simulink model "ah001_full_import"  (R2025b)
settings: Solver=VariableStepAuto  StartTime=0.0  StopTime=10.0  RelTol=1e-3
model workspace: external: MATLAB File C:\Users\Ben\Documents\GitHub\Bipedal_Robot\Neuromechanical_Models\AH001_Simscape_Repair\cad\export\ah001_full_DataFile.m (data not in the file)
undefined symbols (not defined in the file or in its folder): smiData, X, Y, Z
libraries: sm_lib x373, nesl_utility x1
(part 2 of 7)

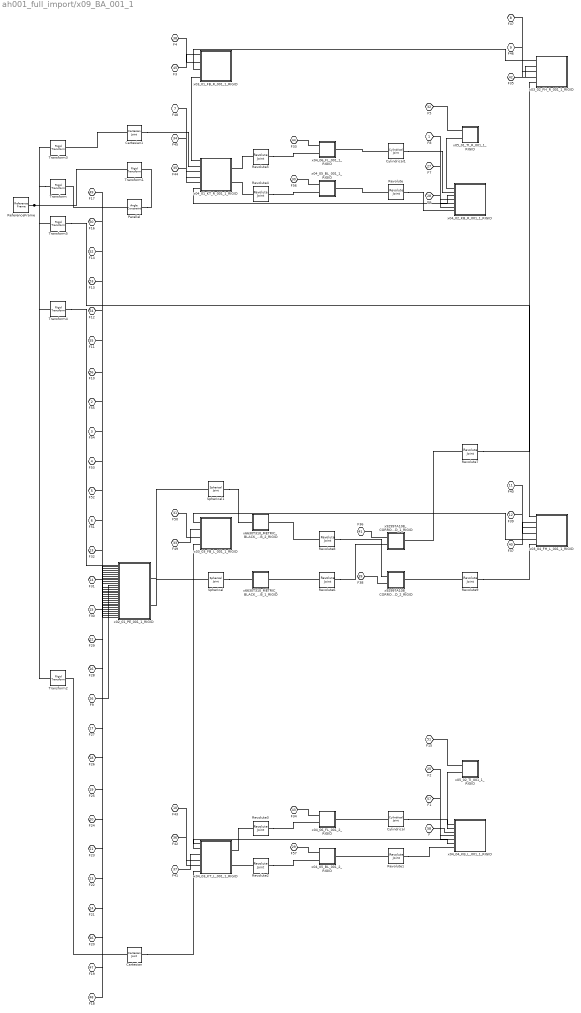
== system ah001_full_import/x09_BA_001_1 ==
  Cartesian : sm_lib/Joints/Cartesian Joint  JointMode=Normal  CompositeWrenchDir=FollowerOnBase  CompositeWrenchFrame=BaseFrame  SenseConstraintForce=off  SenseConstraintTorque=off  SenseTotalForce=off  SenseTotalTorque=off  PxPositionTargetSpecify=on  PxPositionTargetPriority=Low  PxPositionTargetValue=smiData.CartesianJoint(1).Px.Pos  PxPositionTargetValueUnits=m  PxVelocityTargetSpecify=off  PxVelocityTargetPriority=High  PxVelocityTargetValue=0  PxVelocityTargetValueUnits=m/s  PxEquilibriumPosition=0  PxEquilibriumPositionUnits=m  PxSpringStiffness=0  PxSpringStiffnessUnits=N/m  PxDampingCoefficient=0  PxDampingCoefficientUnits=N/(m/s)  PxLowerLimitSpecify=off  PxLowerLimitBound=-1  PxLowerLimitBoundUnits=m  PxLowerLimitStiffness=1e6  PxLowerLimitStiffnessUnits=N/m  PxLowerLimitDamping=1e3  PxLowerLimitDampingUnits=N/(m/s)  PxLowerLimitTransitionRegionWidth=1e-4  PxLowerLimitTransitionRegionWidthUnits=m  PxUpperLimitSpecify=off  PxUpperLimitBound=1  PxUpperLimitBoundUnits=m  PxUpperLimitStiffness=1e6  PxUpperLimitStiffnessUnits=N/m  PxUpperLimitDamping=1e3  PxUpperLimitDampingUnits=N/(m/s)  PxUpperLimitTransitionRegionWidth=1e-4  PxUpperLimitTransitionRegionWidthUnits=m  PxTorqueActuationMode=NoTorque  PxMotionActuationMode=ComputedMotion  PxSensePosition=off  PxSenseVelocity=off  PxSenseAcceleration=off  PxSenseTorqueForce=off  PxSenseLowerLimitTorqueForce=off  PxSenseUpperLimitTorqueForce=off  PyPositionTargetSpecify=on  PyPositionTargetPriority=Low  PyPositionTargetValue=smiData.CartesianJoint(1).Py.Pos  PyPositionTargetValueUnits=m  PyVelocityTargetSpecify=off  PyVelocityTargetPriority=High  PyVelocityTargetValue=0  PyVelocityTargetValueUnits=m/s  PyEquilibriumPosition=0  PyEquilibriumPositionUnits=m  PySpringStiffness=0  PySpringStiffnessUnits=N/m  PyDampingCoefficient=0  PyDampingCoefficientUnits=N/(m/s)  PyLowerLimitSpecify=off  PyLowerLimitBound=-1  PyLowerLimitBoundUnits=m  PyLowerLimitStiffness=1e6  PyLowerLimitStiffnessUnits=N/m  PyLowerLimitDamping=1e3  PyLowerLimitDampingUnits=N/(m/s)  PyLowerLimitTransitionRegionWidth=1e-4  PyLowerLimitTransitionRegionWidthUnits=m  PyUpperLimitSpecify=off  PyUpperLimitBound=1  PyUpperLimitBoundUnits=m  PyUpperLimitStiffness=1e6  PyUpperLimitStiffnessUnits=N/m  PyUpperLimitDamping=1e3  PyUpperLimitDampingUnits=N/(m/s)  PyUpperLimitTransitionRegionWidth=1e-4  PyUpperLimitTransitionRegionWidthUnits=m  PyTorqueActuationMode=NoTorque  PyMotionActuationMode=ComputedMotion  PySensePosition=off  PySenseVelocity=off  PySenseAcceleration=off  PySenseTorqueForce=off  PySenseLowerLimitTorqueForce=off  PySenseUpperLimitTorqueForce=off  PzPositionTargetSpecify=on  PzPositionTargetPriority=Low  PzPositionTargetValue=smiData.CartesianJoint(1).Pz.Pos  PzPositionTargetValueUnits=m  PzVelocityTargetSpecify=off  PzVelocityTargetPriority=High  PzVelocityTargetValue=0  PzVelocityTargetValueUnits=m/s  PzEquilibriumPosition=0  PzEquilibriumPositionUnits=m  PzSpringStiffness=0  PzSpringStiffnessUnits=N/m  PzDampingCoefficient=0  PzDampingCoefficientUnits=N/(m/s)  PzLowerLimitSpecify=off  PzLowerLimitBound=-1  PzLowerLimitBoundUnits=m  PzLowerLimitStiffness=1e6  PzLowerLimitStiffnessUnits=N/m  PzLowerLimitDamping=1e3  PzLowerLimitDampingUnits=N/(m/s)  PzLowerLimitTransitionRegionWidth=1e-4  PzLowerLimitTransitionRegionWidthUnits=m  PzUpperLimitSpecify=off  PzUpperLimitBound=1  PzUpperLimitBoundUnits=m  PzUpperLimitStiffness=1e6  PzUpperLimitStiffnessUnits=N/m  PzUpperLimitDamping=1e3  PzUpperLimitDampingUnits=N/(m/s)  PzUpperLimitTransitionRegionWidth=1e-4  PzUpperLimitTransitionRegionWidthUnits=m  PzTorqueActuationMode=NoTorque  PzMotionActuationMode=ComputedMotion  PzSensePosition=off  PzSenseVelocity=off  PzSenseAcceleration=off  PzSenseTorqueForce=off  PzSenseLowerLimitTorqueForce=off  PzSenseUpperLimitTorqueForce=off
  Cartesian1 : sm_lib/Joints/Cartesian Joint  JointMode=Normal  CompositeWrenchDir=FollowerOnBase  CompositeWrenchFrame=BaseFrame  SenseConstraintForce=off  SenseConstraintTorque=off  SenseTotalForce=off  SenseTotalTorque=off  PxPositionTargetSpecify=off  PxPositionTargetPriority=High  PxPositionTargetValue=0  PxPositionTargetValueUnits=m  PxVelocityTargetSpecify=off  PxVelocityTargetPriority=High  PxVelocityTargetValue=0  PxVelocityTargetValueUnits=m/s  PxEquilibriumPosition=0  PxEquilibriumPositionUnits=m  PxSpringStiffness=0  PxSpringStiffnessUnits=N/m  PxDampingCoefficient=0  PxDampingCoefficientUnits=N/(m/s)  PxLowerLimitSpecify=off  PxLowerLimitBound=-1  PxLowerLimitBoundUnits=m  PxLowerLimitStiffness=1e6  PxLowerLimitStiffnessUnits=N/m  PxLowerLimitDamping=1e3  PxLowerLimitDampingUnits=N/(m/s)  PxLowerLimitTransitionRegionWidth=1e-4  PxLowerLimitTransitionRegionWidthUnits=m  PxUpperLimitSpecify=off  PxUpperLimitBound=1  PxUpperLimitBoundUnits=m  PxUpperLimitStiffness=1e6  PxUpperLimitStiffnessUnits=N/m  PxUpperLimitDamping=1e3  PxUpperLimitDampingUnits=N/(m/s)  PxUpperLimitTransitionRegionWidth=1e-4  PxUpperLimitTransitionRegionWidthUnits=m  PxTorqueActuationMode=NoTorque  PxMotionActuationMode=ComputedMotion  PxSensePosition=off  PxSenseVelocity=off  PxSenseAcceleration=off  PxSenseTorqueForce=off  PxSenseLowerLimitTorqueForce=off  PxSenseUpperLimitTorqueForce=off  PyPositionTargetSpecify=off  PyPositionTargetPriority=High  PyPositionTargetValue=0  PyPositionTargetValueUnits=m  PyVelocityTargetSpecify=off  PyVelocityTargetPriority=High  PyVelocityTargetValue=0  PyVelocityTargetValueUnits=m/s  PyEquilibriumPosition=0  PyEquilibriumPositionUnits=m  PySpringStiffness=0  PySpringStiffnessUnits=N/m  PyDampingCoefficient=0  PyDampingCoefficientUnits=N/(m/s)  PyLowerLimitSpecify=off  PyLowerLimitBound=-1  PyLowerLimitBoundUnits=m  PyLowerLimitStiffness=1e6  PyLowerLimitStiffnessUnits=N/m  PyLowerLimitDamping=1e3  PyLowerLimitDampingUnits=N/(m/s)  PyLowerLimitTransitionRegionWidth=1e-4  PyLowerLimitTransitionRegionWidthUnits=m  PyUpperLimitSpecify=off  PyUpperLimitBound=1  PyUpperLimitBoundUnits=m  PyUpperLimitStiffness=1e6  PyUpperLimitStiffnessUnits=N/m  PyUpperLimitDamping=1e3  PyUpperLimitDampingUnits=N/(m/s)  PyUpperLimitTransitionRegionWidth=1e-4  PyUpperLimitTransitionRegionWidthUnits=m  PyTorqueActuationMode=NoTorque  PyMotionActuationMode=ComputedMotion  PySensePosition=off  PySenseVelocity=off  PySenseAcceleration=off  PySenseTorqueForce=off  PySenseLowerLimitTorqueForce=off  PySenseUpperLimitTorqueForce=off  PzPositionTargetSpecify=off  PzPositionTargetPriority=High  PzPositionTargetValue=0  PzPositionTargetValueUnits=m  PzVelocityTargetSpecify=off  PzVelocityTargetPriority=High  PzVelocityTargetValue=0  PzVelocityTargetValueUnits=m/s  PzEquilibriumPosition=0  PzEquilibriumPositionUnits=m  PzSpringStiffness=0  PzSpringStiffnessUnits=N/m  PzDampingCoefficient=0  PzDampingCoefficientUnits=N/(m/s)  PzLowerLimitSpecify=off  PzLowerLimitBound=-1  PzLowerLimitBoundUnits=m  PzLowerLimitStiffness=1e6  PzLowerLimitStiffnessUnits=N/m  PzLowerLimitDamping=1e3  PzLowerLimitDampingUnits=N/(m/s)  PzLowerLimitTransitionRegionWidth=1e-4  PzLowerLimitTransitionRegionWidthUnits=m  PzUpperLimitSpecify=off  PzUpperLimitBound=1  PzUpperLimitBoundUnits=m  PzUpperLimitStiffness=1e6  PzUpperLimitStiffnessUnits=N/m  PzUpperLimitDamping=1e3  PzUpperLimitDampingUnits=N/(m/s)  PzUpperLimitTransitionRegionWidth=1e-4  PzUpperLimitTransitionRegionWidthUnits=m  PzTorqueActuationMode=NoTorque  PzMotionActuationMode=ComputedMotion  PzSensePosition=off  PzSenseVelocity=off  PzSenseAcceleration=off  PzSenseTorqueForce=off  PzSenseLowerLimitTorqueForce=off  PzSenseUpperLimitTorqueForce=off
  Cylindrical : sm_lib/Joints/Cylindrical Joint  JointMode=Normal  CompositeWrenchDir=FollowerOnBase  CompositeWrenchFrame=BaseFrame  SenseConstraintForce=off  SenseConstraintTorque=off  SenseTotalForce=off  SenseTotalTorque=off  RzPositionTargetSpecify=off  RzPositionTargetPriority=High  RzPositionTargetValue=0  RzPositionTargetValueUnits=deg  RzVelocityTargetSpecify=off  RzVelocityTargetPriority=High  RzVelocityTargetValue=0  RzVelocityTargetValueUnits=deg/s  RzEquilibriumPosition=0  RzEquilibriumPositionUnits=deg  RzSpringStiffness=0  RzSpringStiffnessUnits=N*m/deg  RzDampingCoefficient=0  RzDampingCoefficientUnits=N*m/(deg/s)  RzLowerLimitSpecify=off  RzLowerLimitBound=-90  RzLowerLimitBoundUnits=deg  RzLowerLimitStiffness=1e4  RzLowerLimitStiffnessUnits=N*m/deg  RzLowerLimitDamping=10  RzLowerLimitDampingUnits=N*m/(deg/s)  RzLowerLimitTransitionRegionWidth=0.1  RzLowerLimitTransitionRegionWidthUnits=deg  RzUpperLimitSpecify=off  RzUpperLimitBound=90  RzUpperLimitBoundUnits=deg  RzUpperLimitStiffness=1e4  RzUpperLimitStiffnessUnits=N*m/deg  RzUpperLimitDamping=10  RzUpperLimitDampingUnits=N*m/(deg/s)  RzUpperLimitTransitionRegionWidth=0.1  RzUpperLimitTransitionRegionWidthUnits=deg  RzTorqueActuationMode=NoTorque  RzMotionActuationMode=ComputedMotion  RzSensePosition=off  RzSenseVelocity=off  RzSenseAcceleration=off  RzSenseTorqueForce=off  RzSenseLowerLimitTorqueForce=off  RzSenseUpperLimitTorqueForce=off  PzPositionTargetSpecify=off  PzPositionTargetPriority=High  PzPositionTargetValue=0  PzPositionTargetValueUnits=m  PzVelocityTargetSpecify=off  PzVelocityTargetPriority=High  PzVelocityTargetValue=0  PzVelocityTargetValueUnits=m/s  PzEquilibriumPosition=0  PzEquilibriumPositionUnits=m  PzSpringStiffness=0  PzSpringStiffnessUnits=N/m  PzDampingCoefficient=0  PzDampingCoefficientUnits=N/(m/s)  PzLowerLimitSpecify=off  PzLowerLimitBound=-1  PzLowerLimitBoundUnits=m  PzLowerLimitStiffness=1e6  PzLowerLimitStiffnessUnits=N/m  PzLowerLimitDamping=1e3  PzLowerLimitDampingUnits=N/(m/s)  PzLowerLimitTransitionRegionWidth=1e-4  PzLowerLimitTransitionRegionWidthUnits=m  PzUpperLimitSpecify=off  PzUpperLimitBound=1  PzUpperLimitBoundUnits=m  PzUpperLimitStiffness=1e6  PzUpperLimitStiffnessUnits=N/m  PzUpperLimitDamping=1e3  PzUpperLimitDampingUnits=N/(m/s)  PzUpperLimitTransitionRegionWidth=1e-4  PzUpperLimitTransitionRegionWidthUnits=m  PzTorqueActuationMode=NoTorque  PzMotionActuationMode=ComputedMotion  PzSensePosition=off  PzSenseVelocity=off  PzSenseAcceleration=off  PzSenseTorqueForce=off  PzSenseLowerLimitTorqueForce=off  PzSenseUpperLimitTorqueForce=off
  Cylindrical1 : sm_lib/Joints/Cylindrical Joint  JointMode=Normal  CompositeWrenchDir=FollowerOnBase  CompositeWrenchFrame=BaseFrame  SenseConstraintForce=off  SenseConstraintTorque=off  SenseTotalForce=off  SenseTotalTorque=off  RzPositionTargetSpecify=off  RzPositionTargetPriority=High  RzPositionTargetValue=0  RzPositionTargetValueUnits=deg  RzVelocityTargetSpecify=off  RzVelocityTargetPriority=High  RzVelocityTargetValue=0  RzVelocityTargetValueUnits=deg/s  RzEquilibriumPosition=0  RzEquilibriumPositionUnits=deg  RzSpringStiffness=0  RzSpringStiffnessUnits=N*m/deg  RzDampingCoefficient=0  RzDampingCoefficientUnits=N*m/(deg/s)  RzLowerLimitSpecify=off  RzLowerLimitBound=-90  RzLowerLimitBoundUnits=deg  RzLowerLimitStiffness=1e4  RzLowerLimitStiffnessUnits=N*m/deg  RzLowerLimitDamping=10  RzLowerLimitDampingUnits=N*m/(deg/s)  RzLowerLimitTransitionRegionWidth=0.1  RzLowerLimitTransitionRegionWidthUnits=deg  RzUpperLimitSpecify=off  RzUpperLimitBound=90  RzUpperLimitBoundUnits=deg  RzUpperLimitStiffness=1e4  RzUpperLimitStiffnessUnits=N*m/deg  RzUpperLimitDamping=10  RzUpperLimitDampingUnits=N*m/(deg/s)  RzUpperLimitTransitionRegionWidth=0.1  RzUpperLimitTransitionRegionWidthUnits=deg  RzTorqueActuationMode=NoTorque  RzMotionActuationMode=ComputedMotion  RzSensePosition=off  RzSenseVelocity=off  RzSenseAcceleration=off  RzSenseTorqueForce=off  RzSenseLowerLimitTorqueForce=off  RzSenseUpperLimitTorqueForce=off  PzPositionTargetSpecify=off  PzPositionTargetPriority=High  PzPositionTargetValue=0  PzPositionTargetValueUnits=m  PzVelocityTargetSpecify=off  PzVelocityTargetPriority=High  PzVelocityTargetValue=0  PzVelocityTargetValueUnits=m/s  PzEquilibriumPosition=0  PzEquilibriumPositionUnits=m  PzSpringStiffness=0  PzSpringStiffnessUnits=N/m  PzDampingCoefficient=0  PzDampingCoefficientUnits=N/(m/s)  PzLowerLimitSpecify=off  PzLowerLimitBound=-1  PzLowerLimitBoundUnits=m  PzLowerLimitStiffness=1e6  PzLowerLimitStiffnessUnits=N/m  PzLowerLimitDamping=1e3  PzLowerLimitDampingUnits=N/(m/s)  PzLowerLimitTransitionRegionWidth=1e-4  PzLowerLimitTransitionRegionWidthUnits=m  PzUpperLimitSpecify=off  PzUpperLimitBound=1  PzUpperLimitBoundUnits=m  PzUpperLimitStiffness=1e6  PzUpperLimitStiffnessUnits=N/m  PzUpperLimitDamping=1e3  PzUpperLimitDampingUnits=N/(m/s)  PzUpperLimitTransitionRegionWidth=1e-4  PzUpperLimitTransitionRegionWidthUnits=m  PzTorqueActuationMode=NoTorque  PzMotionActuationMode=ComputedMotion  PzSensePosition=off  PzSenseVelocity=off  PzSenseAcceleration=off  PzSenseTorqueForce=off  PzSenseLowerLimitTorqueForce=off  PzSenseUpperLimitTorqueForce=off
  Parallel : sm_lib/Constraints/Angle Constraint  ConstraintType=Parallel  Angle=45  AngleUnits=deg  WrenchDir=FollowerOnBase  WrenchFrame=BaseFrame  SenseTorque=off  SenseSignedTorqueMagnitude=off
  ReferenceFrame : sm_lib/Frames and Transforms/Reference Frame
  Revolute : sm_lib/Joints/Revolute Joint  JointMode=Normal  CompositeWrenchDir=FollowerOnBase  CompositeWrenchFrame=BaseFrame  SenseConstraintForce=off  SenseConstraintTorque=off  SenseTotalForce=off  SenseTotalTorque=off  PositionTargetSpecify=on  PositionTargetPriority=Low  PositionTargetValue=smiData.RevoluteJoint(1).Rz.Pos  PositionTargetValueUnits=deg  VelocityTargetSpecify=off  VelocityTargetPriority=High  VelocityTargetValue=0  VelocityTargetValueUnits=deg/s  EquilibriumPosition=0  EquilibriumPositionUnits=deg  SpringStiffness=0  SpringStiffnessUnits=N*m/deg  DampingCoefficient=0  DampingCoefficientUnits=N*m/(deg/s)  LowerLimitSpecify=off  LowerLimitBound=-90  LowerLimitBoundUnits=deg  LowerLimitStiffness=1e4  LowerLimitStiffnessUnits=N*m/deg  LowerLimitDamping=10  LowerLimitDampingUnits=N*m/(deg/s)  LowerLimitTransitionRegionWidth=0.1  LowerLimitTransitionRegionWidthUnits=deg  UpperLimitSpecify=off  UpperLimitBound=90  UpperLimitBoundUnits=deg  UpperLimitStiffness=1e4  UpperLimitStiffnessUnits=N*m/deg  UpperLimitDamping=10  UpperLimitDampingUnits=N*m/(deg/s)  UpperLimitTransitionRegionWidth=0.1  UpperLimitTransitionRegionWidthUnits=deg  TorqueActuationMode=NoTorque  MotionActuationMode=ComputedMotion  SensePosition=off  SenseVelocity=off  SenseAcceleration=off  SenseTorqueForce=off  SenseLowerLimitTorqueForce=off  SenseUpperLimitTorqueForce=off
  Revolute1 : sm_lib/Joints/Revolute Joint  JointMode=Normal  CompositeWrenchDir=FollowerOnBase  CompositeWrenchFrame=BaseFrame  SenseConstraintForce=off  SenseConstraintTorque=off  SenseTotalForce=off  SenseTotalTorque=off  PositionTargetSpecify=on  PositionTargetPriority=Low  PositionTargetValue=smiData.RevoluteJoint(2).Rz.Pos  PositionTargetValueUnits=deg  VelocityTargetSpecify=off  VelocityTargetPriority=High  VelocityTargetValue=0  VelocityTargetValueUnits=deg/s  EquilibriumPosition=0  EquilibriumPositionUnits=deg  SpringStiffness=0  SpringStiffnessUnits=N*m/deg  DampingCoefficient=0  DampingCoefficientUnits=N*m/(deg/s)  LowerLimitSpecify=off  LowerLimitBound=-90  LowerLimitBoundUnits=deg  LowerLimitStiffness=1e4  LowerLimitStiffnessUnits=N*m/deg  LowerLimitDamping=10  LowerLimitDampingUnits=N*m/(deg/s)  LowerLimitTransitionRegionWidth=0.1  LowerLimitTransitionRegionWidthUnits=deg  UpperLimitSpecify=off  UpperLimitBound=90  UpperLimitBoundUnits=deg  UpperLimitStiffness=1e4  UpperLimitStiffnessUnits=N*m/deg  UpperLimitDamping=10  UpperLimitDampingUnits=N*m/(deg/s)  UpperLimitTransitionRegionWidth=0.1  UpperLimitTransitionRegionWidthUnits=deg  TorqueActuationMode=NoTorque  MotionActuationMode=ComputedMotion  SensePosition=off  SenseVelocity=off  SenseAcceleration=off  SenseTorqueForce=off  SenseLowerLimitTorqueForce=off  SenseUpperLimitTorqueForce=off
  Revolute2 : sm_lib/Joints/Revolute Joint  JointMode=Normal  CompositeWrenchDir=FollowerOnBase  CompositeWrenchFrame=BaseFrame  SenseConstraintForce=off  SenseConstraintTorque=off  SenseTotalForce=off  SenseTotalTorque=off  PositionTargetSpecify=off  PositionTargetPriority=High  PositionTargetValue=0  PositionTargetValueUnits=deg  VelocityTargetSpecify=off  VelocityTargetPriority=High  VelocityTargetValue=0  VelocityTargetValueUnits=deg/s  EquilibriumPosition=0  EquilibriumPositionUnits=deg  SpringStiffness=0  SpringStiffnessUnits=N*m/deg  DampingCoefficient=0  DampingCoefficientUnits=N*m/(deg/s)  LowerLimitSpecify=off  LowerLimitBound=-90  LowerLimitBoundUnits=deg  LowerLimitStiffness=1e4  LowerLimitStiffnessUnits=N*m/deg  LowerLimitDamping=10  LowerLimitDampingUnits=N*m/(deg/s)  LowerLimitTransitionRegionWidth=0.1  LowerLimitTransitionRegionWidthUnits=deg  UpperLimitSpecify=off  UpperLimitBound=90  UpperLimitBoundUnits=deg  UpperLimitStiffness=1e4  UpperLimitStiffnessUnits=N*m/deg  UpperLimitDamping=10  UpperLimitDampingUnits=N*m/(deg/s)  UpperLimitTransitionRegionWidth=0.1  UpperLimitTransitionRegionWidthUnits=deg  TorqueActuationMode=NoTorque  MotionActuationMode=ComputedMotion  SensePosition=off  SenseVelocity=off  SenseAcceleration=off  SenseTorqueForce=off  SenseLowerLimitTorqueForce=off  SenseUpperLimitTorqueForce=off
  Revolute3 : sm_lib/Joints/Revolute Joint  JointMode=Normal  CompositeWrenchDir=FollowerOnBase  CompositeWrenchFrame=BaseFrame  SenseConstraintForce=off  SenseConstraintTorque=off  SenseTotalForce=off  SenseTotalTorque=off  PositionTargetSpecify=on  PositionTargetPriority=Low  PositionTargetValue=smiData.RevoluteJoint(4).Rz.Pos  PositionTargetValueUnits=deg  VelocityTargetSpecify=off  VelocityTargetPriority=High  VelocityTargetValue=0  VelocityTargetValueUnits=deg/s  EquilibriumPosition=0  EquilibriumPositionUnits=deg  SpringStiffness=0  SpringStiffnessUnits=N*m/deg  DampingCoefficient=0  DampingCoefficientUnits=N*m/(deg/s)  LowerLimitSpecify=off  LowerLimitBound=-90  LowerLimitBoundUnits=deg  LowerLimitStiffness=1e4  LowerLimitStiffnessUnits=N*m/deg  LowerLimitDamping=10  LowerLimitDampingUnits=N*m/(deg/s)  LowerLimitTransitionRegionWidth=0.1  LowerLimitTransitionRegionWidthUnits=deg  UpperLimitSpecify=off  UpperLimitBound=90  UpperLimitBoundUnits=deg  UpperLimitStiffness=1e4  UpperLimitStiffnessUnits=N*m/deg  UpperLimitDamping=10  UpperLimitDampingUnits=N*m/(deg/s)  UpperLimitTransitionRegionWidth=0.1  UpperLimitTransitionRegionWidthUnits=deg  TorqueActuationMode=NoTorque  MotionActuationMode=ComputedMotion  SensePosition=off  SenseVelocity=off  SenseAcceleration=off  SenseTorqueForce=off  SenseLowerLimitTorqueForce=off  SenseUpperLimitTorqueForce=off
  Revolute4 : sm_lib/Joints/Revolute Joint  JointMode=Normal  CompositeWrenchDir=FollowerOnBase  CompositeWrenchFrame=BaseFrame  SenseConstraintForce=off  SenseConstraintTorque=off  SenseTotalForce=off  SenseTotalTorque=off  PositionTargetSpecify=off  PositionTargetPriority=High  PositionTargetValue=0  PositionTargetValueUnits=deg  VelocityTargetSpecify=off  VelocityTargetPriority=High  VelocityTargetValue=0  VelocityTargetValueUnits=deg/s  EquilibriumPosition=0  EquilibriumPositionUnits=deg  SpringStiffness=0  SpringStiffnessUnits=N*m/deg  DampingCoefficient=0  DampingCoefficientUnits=N*m/(deg/s)  LowerLimitSpecify=off  LowerLimitBound=-90  LowerLimitBoundUnits=deg  LowerLimitStiffness=1e4  LowerLimitStiffnessUnits=N*m/deg  LowerLimitDamping=10  LowerLimitDampingUnits=N*m/(deg/s)  LowerLimitTransitionRegionWidth=0.1  LowerLimitTransitionRegionWidthUnits=deg  UpperLimitSpecify=off  UpperLimitBound=90  UpperLimitBoundUnits=deg  UpperLimitStiffness=1e4  UpperLimitStiffnessUnits=N*m/deg  UpperLimitDamping=10  UpperLimitDampingUnits=N*m/(deg/s)  UpperLimitTransitionRegionWidth=0.1  UpperLimitTransitionRegionWidthUnits=deg  TorqueActuationMode=NoTorque  MotionActuationMode=ComputedMotion  SensePosition=off  SenseVelocity=off  SenseAcceleration=off  SenseTorqueForce=off  SenseLowerLimitTorqueForce=off  SenseUpperLimitTorqueForce=off
  Revolute5 : sm_lib/Joints/Revolute Joint  JointMode=Normal  CompositeWrenchDir=FollowerOnBase  CompositeWrenchFrame=BaseFrame  SenseConstraintForce=off  SenseConstraintTorque=off  SenseTotalForce=off  SenseTotalTorque=off  PositionTargetSpecify=on  PositionTargetPriority=Low  PositionTargetValue=smiData.RevoluteJoint(6).Rz.Pos  PositionTargetValueUnits=deg  VelocityTargetSpecify=off  VelocityTargetPriority=High  VelocityTargetValue=0  VelocityTargetValueUnits=deg/s  EquilibriumPosition=0  EquilibriumPositionUnits=deg  SpringStiffness=0  SpringStiffnessUnits=N*m/deg  DampingCoefficient=0  DampingCoefficientUnits=N*m/(deg/s)  LowerLimitSpecify=off  LowerLimitBound=-90  LowerLimitBoundUnits=deg  LowerLimitStiffness=1e4  LowerLimitStiffnessUnits=N*m/deg  LowerLimitDamping=10  LowerLimitDampingUnits=N*m/(deg/s)  LowerLimitTransitionRegionWidth=0.1  LowerLimitTransitionRegionWidthUnits=deg  UpperLimitSpecify=off  UpperLimitBound=90  UpperLimitBoundUnits=deg  UpperLimitStiffness=1e4  UpperLimitStiffnessUnits=N*m/deg  UpperLimitDamping=10  UpperLimitDampingUnits=N*m/(deg/s)  UpperLimitTransitionRegionWidth=0.1  UpperLimitTransitionRegionWidthUnits=deg  TorqueActuationMode=NoTorque  MotionActuationMode=ComputedMotion  SensePosition=off  SenseVelocity=off  SenseAcceleration=off  SenseTorqueForce=off  SenseLowerLimitTorqueForce=off  SenseUpperLimitTorqueForce=off
  Revolute6 : sm_lib/Joints/Revolute Joint  JointMode=Normal  CompositeWrenchDir=FollowerOnBase  CompositeWrenchFrame=BaseFrame  SenseConstraintForce=off  SenseConstraintTorque=off  SenseTotalForce=off  SenseTotalTorque=off  PositionTargetSpecify=on  PositionTargetPriority=Low  PositionTargetValue=smiData.RevoluteJoint(7).Rz.Pos  PositionTargetValueUnits=deg  VelocityTargetSpecify=off  VelocityTargetPriority=High  VelocityTargetValue=0  VelocityTargetValueUnits=deg/s  EquilibriumPosition=0  EquilibriumPositionUnits=deg  SpringStiffness=0  SpringStiffnessUnits=N*m/deg  DampingCoefficient=0  DampingCoefficientUnits=N*m/(deg/s)  LowerLimitSpecify=off  LowerLimitBound=-90  LowerLimitBoundUnits=deg  LowerLimitStiffness=1e4  LowerLimitStiffnessUnits=N*m/deg  LowerLimitDamping=10  LowerLimitDampingUnits=N*m/(deg/s)  LowerLimitTransitionRegionWidth=0.1  LowerLimitTransitionRegionWidthUnits=deg  UpperLimitSpecify=off  UpperLimitBound=90  UpperLimitBoundUnits=deg  UpperLimitStiffness=1e4  UpperLimitStiffnessUnits=N*m/deg  UpperLimitDamping=10  UpperLimitDampingUnits=N*m/(deg/s)  UpperLimitTransitionRegionWidth=0.1  UpperLimitTransitionRegionWidthUnits=deg  TorqueActuationMode=NoTorque  MotionActuationMode=ComputedMotion  SensePosition=off  SenseVelocity=off  SenseAcceleration=off  SenseTorqueForce=off  SenseLowerLimitTorqueForce=off  SenseUpperLimitTorqueForce=off
  Revolute7 : sm_lib/Joints/Revolute Joint  JointMode=Normal  CompositeWrenchDir=FollowerOnBase  CompositeWrenchFrame=BaseFrame  SenseConstraintForce=off  SenseConstraintTorque=off  SenseTotalForce=off  SenseTotalTorque=off  PositionTargetSpecify=on  PositionTargetPriority=Low  PositionTargetValue=smiData.RevoluteJoint(8).Rz.Pos  PositionTargetValueUnits=deg  VelocityTargetSpecify=off  VelocityTargetPriority=High  VelocityTargetValue=0  VelocityTargetValueUnits=deg/s  EquilibriumPosition=0  EquilibriumPositionUnits=deg  SpringStiffness=0  SpringStiffnessUnits=N*m/deg  DampingCoefficient=0  DampingCoefficientUnits=N*m/(deg/s)  LowerLimitSpecify=off  LowerLimitBound=-90  LowerLimitBoundUnits=deg  LowerLimitStiffness=1e4  LowerLimitStiffnessUnits=N*m/deg  LowerLimitDamping=10  LowerLimitDampingUnits=N*m/(deg/s)  LowerLimitTransitionRegionWidth=0.1  LowerLimitTransitionRegionWidthUnits=deg  UpperLimitSpecify=off  UpperLimitBound=90  UpperLimitBoundUnits=deg  UpperLimitStiffness=1e4  UpperLimitStiffnessUnits=N*m/deg  UpperLimitDamping=10  UpperLimitDampingUnits=N*m/(deg/s)  UpperLimitTransitionRegionWidth=0.1  UpperLimitTransitionRegionWidthUnits=deg  TorqueActuationMode=NoTorque  MotionActuationMode=ComputedMotion  SensePosition=off  SenseVelocity=off  SenseAcceleration=off  SenseTorqueForce=off  SenseLowerLimitTorqueForce=off  SenseUpperLimitTorqueForce=off
  Revolute8 : sm_lib/Joints/Revolute Joint  JointMode=Normal  CompositeWrenchDir=FollowerOnBase  CompositeWrenchFrame=BaseFrame  SenseConstraintForce=off  SenseConstraintTorque=off  SenseTotalForce=off  SenseTotalTorque=off  PositionTargetSpecify=on  PositionTargetPriority=Low  PositionTargetValue=smiData.RevoluteJoint(9).Rz.Pos  PositionTargetValueUnits=deg  VelocityTargetSpecify=off  VelocityTargetPriority=High  VelocityTargetValue=0  VelocityTargetValueUnits=deg/s  EquilibriumPosition=0  EquilibriumPositionUnits=deg  SpringStiffness=0  SpringStiffnessUnits=N*m/deg  DampingCoefficient=0  DampingCoefficientUnits=N*m/(deg/s)  LowerLimitSpecify=off  LowerLimitBound=-90  LowerLimitBoundUnits=deg  LowerLimitStiffness=1e4  LowerLimitStiffnessUnits=N*m/deg  LowerLimitDamping=10  LowerLimitDampingUnits=N*m/(deg/s)  LowerLimitTransitionRegionWidth=0.1  LowerLimitTransitionRegionWidthUnits=deg  UpperLimitSpecify=off  UpperLimitBound=90  UpperLimitBoundUnits=deg  UpperLimitStiffness=1e4  UpperLimitStiffnessUnits=N*m/deg  UpperLimitDamping=10  UpperLimitDampingUnits=N*m/(deg/s)  UpperLimitTransitionRegionWidth=0.1  UpperLimitTransitionRegionWidthUnits=deg  TorqueActuationMode=NoTorque  MotionActuationMode=ComputedMotion  SensePosition=off  SenseVelocity=off  SenseAcceleration=off  SenseTorqueForce=off  SenseLowerLimitTorqueForce=off  SenseUpperLimitTorqueForce=off
  Revolute9 : sm_lib/Joints/Revolute Joint  JointMode=Normal  CompositeWrenchDir=FollowerOnBase  CompositeWrenchFrame=BaseFrame  SenseConstraintForce=off  SenseConstraintTorque=off  SenseTotalForce=off  SenseTotalTorque=off  PositionTargetSpecify=on  PositionTargetPriority=Low  PositionTargetValue=smiData.RevoluteJoint(10).Rz.Pos  PositionTargetValueUnits=deg  VelocityTargetSpecify=off  VelocityTargetPriority=High  VelocityTargetValue=0  VelocityTargetValueUnits=deg/s  EquilibriumPosition=0  EquilibriumPositionUnits=deg  SpringStiffness=0  SpringStiffnessUnits=N*m/deg  DampingCoefficient=0  DampingCoefficientUnits=N*m/(deg/s)  LowerLimitSpecify=off  LowerLimitBound=-90  LowerLimitBoundUnits=deg  LowerLimitStiffness=1e4  LowerLimitStiffnessUnits=N*m/deg  LowerLimitDamping=10  LowerLimitDampingUnits=N*m/(deg/s)  LowerLimitTransitionRegionWidth=0.1  LowerLimitTransitionRegionWidthUnits=deg  UpperLimitSpecify=off  UpperLimitBound=90  UpperLimitBoundUnits=deg  UpperLimitStiffness=1e4  UpperLimitStiffnessUnits=N*m/deg  UpperLimitDamping=10  UpperLimitDampingUnits=N*m/(deg/s)  UpperLimitTransitionRegionWidth=0.1  UpperLimitTransitionRegionWidthUnits=deg  TorqueActuationMode=NoTorque  MotionActuationMode=ComputedMotion  SensePosition=off  SenseVelocity=off  SenseAcceleration=off  SenseTorqueForce=off  SenseLowerLimitTorqueForce=off  SenseUpperLimitTorqueForce=off
  Spherical : sm_lib/Joints/Spherical Joint  JointMode=Normal  CompositeWrenchDir=FollowerOnBase  CompositeWrenchFrame=BaseFrame  SenseConstraintForce=off  SenseConstraintTorque=off  SenseTotalForce=off  SenseTotalTorque=off  PositionTargetSpecify=on  PositionTargetPriority=Low  PositionTargetRotationMethod=ArbitraryAxis  PositionTargetFollAlignAxisA=+X  PositionTargetBaseAlignAxisA=+Y  PositionTargetFollAlignAxisB=+Y  PositionTargetBaseAlignAxisB=+Z  PositionTargetRotationStandardAxis=+Z  PositionTargetRotationAngle=smiData.SphericalJoint(1).S.Pos.Angle  PositionTargetRotationAngleUnits=deg  PositionTargetRotationArbitraryAxis=smiData.SphericalJoint(1).S.Pos.Axis  PositionTargetRotationSequenceAxes=FollowerAxes  PositionTargetRotationSequence=XYX  PositionTargetRotationSequenceAngles=[0 0 0]  PositionTargetRotationSequenceAnglesUnits=deg  PositionTargetRotationMatrix=[1 0 0;0 1 0;0 0 1]  PositionTargetQuaternion=[1 0 0 0]  VelocityTargetSpecify=off  VelocityTargetPriority=High  VelocityTargetValue=[0 0 0]  VelocityTargetValueUnits=deg/s  VelocityTargetInFollowerFrame=on  EqPosRotationMethod=None  EqPosFollAlignAxisA=+X  EqPosBaseAlignAxisA=+Y  EqPosFollAlignAxisB=+Y  EqPosBaseAlignAxisB=+Z  EqPosRotationStandardAxis=+Z  EqPosRotationAngle=0  EqPosRotationAngleUnits=deg  EqPosRotationArbitraryAxis=[0 0 1]  EqPosRotationSequenceAxes=FollowerAxes  EqPosRotationSequence=XYX  EqPosRotationSequenceAngles=[0 0 0]  EqPosRotationSequenceAnglesUnits=deg  EqPosRotationMatrix=[1 0 0;0 1 0;0 0 1]  EqPosQuaternion=[1 0 0 0]  SpringStiffness=0  SpringStiffnessUnits=N*m/deg  DampingCoefficient=0  DampingCoefficientUnits=N*m/(deg/s)  LowerLimitSpecify=off  LowerLimitBound=15  LowerLimitBoundUnits=deg  LowerLimitStiffness=1e4  LowerLimitStiffnessUnits=N*m/deg  LowerLimitDamping=10  LowerLimitDampingUnits=N*m/(deg/s)  LowerLimitTransitionRegionWidth=0.1  LowerLimitTransitionRegionWidthUnits=deg  UpperLimitSpecify=off  UpperLimitBound=45  UpperLimitBoundUnits=deg  UpperLimitStiffness=1e4  UpperLimitStiffnessUnits=N*m/deg  UpperLimitDamping=10  UpperLimitDampingUnits=N*m/(deg/s)  UpperLimitTransitionRegionWidth=0.1  UpperLimitTransitionRegionWidthUnits=deg  TorqueActuationMode=NoTorque  ActuateTorqueX=off  ActuateTorqueY=off  ActuateTorqueZ=off  ActuateTorque=off  ActuationFrame=BaseFrame  SensePosition=off  SenseVelocityX=off  SenseVelocityY=off  SenseVelocityZ=off  SenseVelocity=off  SenseAccelerationX=off  SenseAccelerationY=off  SenseAccelerationZ=off  SenseAcceleration=off  SenseLowerLimitTorqueMag=off  SenseUpperLimitTorqueMag=off  SensingFrame=FollowerFrame
  Spherical1 : sm_lib/Joints/Spherical Joint  JointMode=Normal  CompositeWrenchDir=FollowerOnBase  CompositeWrenchFrame=BaseFrame  SenseConstraintForce=off  SenseConstraintTorque=off  SenseTotalForce=off  SenseTotalTorque=off  PositionTargetSpecify=off  PositionTargetPriority=High  PositionTargetRotationMethod=None  PositionTargetFollAlignAxisA=+X  PositionTargetBaseAlignAxisA=+Y  PositionTargetFollAlignAxisB=+Y  PositionTargetBaseAlignAxisB=+Z  PositionTargetRotationStandardAxis=+Z  PositionTargetRotationAngle=0  PositionTargetRotationAngleUnits=deg  PositionTargetRotationArbitraryAxis=[0 0 1]  PositionTargetRotationSequenceAxes=FollowerAxes  PositionTargetRotationSequence=XYX  PositionTargetRotationSequenceAngles=[0 0 0]  PositionTargetRotationSequenceAnglesUnits=deg  PositionTargetRotationMatrix=[1 0 0;0 1 0;0 0 1]  PositionTargetQuaternion=[1 0 0 0]  VelocityTargetSpecify=off  VelocityTargetPriority=High  VelocityTargetValue=[0 0 0]  VelocityTargetValueUnits=deg/s  VelocityTargetInFollowerFrame=on  EqPosRotationMethod=None  EqPosFollAlignAxisA=+X  EqPosBaseAlignAxisA=+Y  EqPosFollAlignAxisB=+Y  EqPosBaseAlignAxisB=+Z  EqPosRotationStandardAxis=+Z  EqPosRotationAngle=0  EqPosRotationAngleUnits=deg  EqPosRotationArbitraryAxis=[0 0 1]  EqPosRotationSequenceAxes=FollowerAxes  EqPosRotationSequence=XYX  EqPosRotationSequenceAngles=[0 0 0]  EqPosRotationSequenceAnglesUnits=deg  EqPosRotationMatrix=[1 0 0;0 1 0;0 0 1]  EqPosQuaternion=[1 0 0 0]  SpringStiffness=0  SpringStiffnessUnits=N*m/deg  DampingCoefficient=0  DampingCoefficientUnits=N*m/(deg/s)  LowerLimitSpecify=off  LowerLimitBound=15  LowerLimitBoundUnits=deg  LowerLimitStiffness=1e4  LowerLimitStiffnessUnits=N*m/deg  LowerLimitDamping=10  LowerLimitDampingUnits=N*m/(deg/s)  LowerLimitTransitionRegionWidth=0.1  LowerLimitTransitionRegionWidthUnits=deg  UpperLimitSpecify=off  UpperLimitBound=45  UpperLimitBoundUnits=deg  UpperLimitStiffness=1e4  UpperLimitStiffnessUnits=N*m/deg  UpperLimitDamping=10  UpperLimitDampingUnits=N*m/(deg/s)  UpperLimitTransitionRegionWidth=0.1  UpperLimitTransitionRegionWidthUnits=deg  TorqueActuationMode=NoTorque  ActuateTorqueX=off  ActuateTorqueY=off  ActuateTorqueZ=off  ActuateTorque=off  ActuationFrame=BaseFrame  SensePosition=off  SenseVelocityX=off  SenseVelocityY=off  SenseVelocityZ=off  SenseVelocity=off  SenseAccelerationX=off  SenseAccelerationY=off  SenseAccelerationZ=off  SenseAcceleration=off  SenseLowerLimitTorqueMag=off  SenseUpperLimitTorqueMag=off  SensingFrame=FollowerFrame
  Transform : sm_lib/Frames and Transforms/Rigid Transform  RotationMethod=ArbitraryAxis  FollAlignAxisA=+X  BaseAlignAxisA=+Y  FollAlignAxisB=+Y  BaseAlignAxisB=+Z  RotationStandardAxis=+Z  RotationAngle=smiData.RigidTransform(21).angle  RotationAngleUnits=rad  RotationArbitraryAxis=smiData.RigidTransform(21).axis  RotationSequenceAxes=FollowerAxes  RotationSequence=XYX  RotationSequenceAngles=[0 0 0]  RotationSequenceAnglesUnits=deg  RotationMatrix=[1 0 0;0 1 0;0 0 1]  Quaternion=[1 0 0 0]  TranslationMethod=Cartesian  TranslationCartesianOffset=smiData.RigidTransform(21).translation  TranslationCartesianOffsetUnits=mm  TranslationStandardAxis=+Z  TranslationStandardOffset=0  TranslationStandardOffsetUnits=m  TranslationROffset=0  TranslationROffsetUnits=m  TranslationThetaOffset=0  TranslationThetaOffsetUnits=deg  TranslationZOffset=0  TranslationZOffsetUnits=m
  Transform1 : sm_lib/Frames and Transforms/Rigid Transform  RotationMethod=ArbitraryAxis  FollAlignAxisA=+X  BaseAlignAxisA=+Y  FollAlignAxisB=+Y  BaseAlignAxisB=+Z  RotationStandardAxis=+Z  RotationAngle=smiData.RigidTransform(22).angle  RotationAngleUnits=rad  RotationArbitraryAxis=smiData.RigidTransform(22).axis  RotationSequenceAxes=FollowerAxes  RotationSequence=XYX  RotationSequenceAngles=[0 0 0]  RotationSequenceAnglesUnits=deg  RotationMatrix=[1 0 0;0 1 0;0 0 1]  Quaternion=[1 0 0 0]  TranslationMethod=Cartesian  TranslationCartesianOffset=smiData.RigidTransform(22).translation  TranslationCartesianOffsetUnits=mm  TranslationStandardAxis=+Z  TranslationStandardOffset=0  TranslationStandardOffsetUnits=m  TranslationROffset=0  TranslationROffsetUnits=m  TranslationThetaOffset=0  TranslationThetaOffsetUnits=deg  TranslationZOffset=0  TranslationZOffsetUnits=m
  Transform2 : sm_lib/Frames and Transforms/Rigid Transform  RotationMethod=ArbitraryAxis  FollAlignAxisA=+X  BaseAlignAxisA=+Y  FollAlignAxisB=+Y  BaseAlignAxisB=+Z  RotationStandardAxis=+Z  RotationAngle=smiData.RigidTransform(23).angle  RotationAngleUnits=rad  RotationArbitraryAxis=smiData.RigidTransform(23).axis  RotationSequenceAxes=FollowerAxes  RotationSequence=XYX  RotationSequenceAngles=[0 0 0]  RotationSequenceAnglesUnits=deg  RotationMatrix=[1 0 0;0 1 0;0 0 1]  Quaternion=[1 0 0 0]  TranslationMethod=Cartesian  TranslationCartesianOffset=smiData.RigidTransform(23).translation  TranslationCartesianOffsetUnits=mm  TranslationStandardAxis=+Z  TranslationStandardOffset=0  TranslationStandardOffsetUnits=m  TranslationROffset=0  TranslationROffsetUnits=m  TranslationThetaOffset=0  TranslationThetaOffsetUnits=deg  TranslationZOffset=0  TranslationZOffsetUnits=m
  Transform3 : sm_lib/Frames and Transforms/Rigid Transform  RotationMethod=ArbitraryAxis  FollAlignAxisA=+X  BaseAlignAxisA=+Y  FollAlignAxisB=+Y  BaseAlignAxisB=+Z  RotationStandardAxis=+Z  RotationAngle=smiData.RigidTransform(37).angle  RotationAngleUnits=rad  RotationArbitraryAxis=smiData.RigidTransform(37).axis  RotationSequenceAxes=FollowerAxes  RotationSequence=XYX  RotationSequenceAngles=[0 0 0]  RotationSequenceAnglesUnits=deg  RotationMatrix=[1 0 0;0 1 0;0 0 1]  Quaternion=[1 0 0 0]  TranslationMethod=Cartesian  TranslationCartesianOffset=smiData.RigidTransform(37).translation  TranslationCartesianOffsetUnits=mm  TranslationStandardAxis=+Z  TranslationStandardOffset=0  TranslationStandardOffsetUnits=m  TranslationROffset=0  TranslationROffsetUnits=m  TranslationThetaOffset=0  TranslationThetaOffsetUnits=deg  TranslationZOffset=0  TranslationZOffsetUnits=m
  Transform4 : sm_lib/Frames and Transforms/Rigid Transform  RotationMethod=ArbitraryAxis  FollAlignAxisA=+X  BaseAlignAxisA=+Y  FollAlignAxisB=+Y  BaseAlignAxisB=+Z  RotationStandardAxis=+Z  RotationAngle=smiData.RigidTransform(167).angle  RotationAngleUnits=rad  RotationArbitraryAxis=smiData.RigidTransform(167).axis  RotationSequenceAxes=FollowerAxes  RotationSequence=XYX  RotationSequenceAngles=[0 0 0]  RotationSequenceAnglesUnits=deg  RotationMatrix=[1 0 0;0 1 0;0 0 1]  Quaternion=[1 0 0 0]  TranslationMethod=Cartesian  TranslationCartesianOffset=smiData.RigidTransform(167).translation  TranslationCartesianOffsetUnits=mm  TranslationStandardAxis=+Z  TranslationStandardOffset=0  TranslationStandardOffsetUnits=m  TranslationROffset=0  TranslationROffsetUnits=m  TranslationThetaOffset=0  TranslationThetaOffsetUnits=deg  TranslationZOffset=0  TranslationZOffsetUnits=m
  Transform5 : sm_lib/Frames and Transforms/Rigid Transform  RotationMethod=ArbitraryAxis  FollAlignAxisA=+X  BaseAlignAxisA=+Y  FollAlignAxisB=+Y  BaseAlignAxisB=+Z  RotationStandardAxis=+Z  RotationAngle=smiData.RigidTransform(168).angle  RotationAngleUnits=rad  RotationArbitraryAxis=smiData.RigidTransform(168).axis  RotationSequenceAxes=FollowerAxes  RotationSequence=XYX  RotationSequenceAngles=[0 0 0]  RotationSequenceAnglesUnits=deg  RotationMatrix=[1 0 0;0 1 0;0 0 1]  Quaternion=[1 0 0 0]  TranslationMethod=Cartesian  TranslationCartesianOffset=smiData.RigidTransform(168).translation  TranslationCartesianOffsetUnits=mm  TranslationStandardAxis=+Z  TranslationStandardOffset=0  TranslationStandardOffsetUnits=m  TranslationROffset=0  TranslationROffsetUnits=m  TranslationThetaOffset=0  TranslationThetaOffsetUnits=deg  TranslationZOffset=0  TranslationZOffsetUnits=m
  x02_01_PE_001_1_RIGID : Subsystem
  x03_01_FB_R_001_1_RIGID : Subsystem
  x03_02_FH_R_001_1_RIGID : Subsystem
  x03_03_FB_L_001_1_RIGID : Subsystem
  x03_04_FH_L_001_1_RIGID : Subsystem
  x04_01_KT_R_001_1_RIGID : Subsystem
  x04_02_KB_R_001_1_RIGID : Subsystem
  x04_03_KT_L_001_1_RIGID : Subsystem
  x04_04_KB_L_001_1_RIGID : Subsystem
  x04_05_BL_001_1_RIGID : Subsystem
  x04_05_BL_001_2_RIGID : Subsystem
  x04_06_FL_001_1_RIGID : Subsystem
  x04_06_FL_001_2_RIGID : Subsystem
  x05_01_TI_R_001_1_RIGID : Subsystem
  x05_02_TI_001_1_RIGID : Subsystem
  x6630T310_METRIC_BLACK_POLYPROPYLENE_BALL_KNOB_1_RIGID : Subsystem
  x6630T310_METRIC_BLACK_POLYPROPYLENE_BALL_KNOB_2_RIGID : Subsystem
  x92997A108_CORROSION_RESISTANT_SETUP_STUD_1_RIGID : Subsystem
  x92997A108_CORROSION_RESISTANT_SETUP_STUD_2_RIGID : Subsystem
  F8 : PMIOPort  Side=Left
  F55 : PMIOPort  Port=2  Side=Left
  F54 : PMIOPort  Port=3  Side=Left
  F53 : PMIOPort  Port=4  Side=Left
  F52 : PMIOPort  Port=5  Side=Left
  F51 : PMIOPort  Port=6  Side=Left
  F48 : PMIOPort  Port=7  Side=Left
  F47 : PMIOPort  Port=8  Side=Left
  F46 : PMIOPort  Port=9  Side=Left
  F43 : PMIOPort  Port=10  Side=Left
  F40 : PMIOPort  Port=11  Side=Left
  F39 : PMIOPort  Port=12  Side=Left
  F32 : PMIOPort  Port=13  Side=Left
  F31 : PMIOPort  Port=14  Side=Left
  F30 : PMIOPort  Port=15  Side=Left
  F28 : PMIOPort  Port=16  Side=Left
  F27 : PMIOPort  Port=17  Side=Left
  F26 : PMIOPort  Port=18  Side=Left
  F25 : PMIOPort  Port=19  Side=Left
  F24 : PMIOPort  Port=20  Side=Left
  F23 : PMIOPort  Port=21  Side=Left
  F29 : PMIOPort  Port=22  Side=Left
  F22 : PMIOPort  Port=23  Side=Left
  F21 : PMIOPort  Port=24  Side=Left
  F2 : PMIOPort  Port=25  Side=Left
  F9 : PMIOPort  Port=26  Side=Right
  F7 : PMIOPort  Port=27  Side=Right
  F6 : PMIOPort  Port=28  Side=Right
  F57 : PMIOPort  Port=29  Side=Right
  F56 : PMIOPort  Port=30  Side=Right
  F50 : PMIOPort  Port=31  Side=Right
  F5 : PMIOPort  Port=32  Side=Right
  F49 : PMIOPort  Port=33  Side=Right
  F45 : PMIOPort  Port=34  Side=Right
  F44 : PMIOPort  Port=35  Side=Right
  F42 : PMIOPort  Port=36  Side=Right
  F41 : PMIOPort  Port=37  Side=Right
  F4 : PMIOPort  Port=38  Side=Right
  F38 : PMIOPort  Port=39  Side=Right
  F37 : PMIOPort  Port=40  Side=Right
  F36 : PMIOPort  Port=41  Side=Right
  F35 : PMIOPort  Port=42  Side=Right
  F34 : PMIOPort  Port=43  Side=Right
  F33 : PMIOPort  Port=44  Side=Right
  F3 : PMIOPort  Port=45  Side=Right
  F20 : PMIOPort  Port=46  Side=Right
  F19 : PMIOPort  Port=47  Side=Right
  F18 : PMIOPort  Port=48  Side=Right
  F17 : PMIOPort  Port=49  Side=Right
  F16 : PMIOPort  Port=50  Side=Right
  F15 : PMIOPort  Port=51  Side=Right
  F14 : PMIOPort  Port=52  Side=Right
  F13 : PMIOPort  Port=53  Side=Right
  F12 : PMIOPort  Port=54  Side=Right
  F11 : PMIOPort  Port=55  Side=Right
  F10 : PMIOPort  Port=56  Side=Right
  F1 : PMIOPort  Port=57  Side=Right
  F : PMIOPort  Port=58  Side=Right
  connections:
  Revolute/LConn1 -- x04_05_BL_001_1_RIGID/RConn1
  Revolute/RConn1 -- x04_02_KB_R_001_1_RIGID/LConn7
  Spherical/RConn1 -- x6630T310_METRIC_BLACK_POLYPROPYLENE_BALL_KNOB_1_RIGID/LConn1
  x04_05_BL_001_2_RIGID/LConn1 -- F57/RConn1
  Transform4/RConn1 -- x02_01_PE_001_1_RIGID/LConn1
  Transform5/RConn1 -- x03_04_FH_L_001_1_RIGID/LConn1
  Spherical1/LConn1 -- x02_01_PE_001_1_RIGID/RConn1
  Spherical1/RConn1 -- x6630T310_METRIC_BLACK_POLYPROPYLENE_BALL_KNOB_2_RIGID/LConn1
  Cylindrical/LConn1 -- x04_06_FL_001_2_RIGID/RConn1
  Cylindrical/RConn1 -- x04_04_KB_L_001_1_RIGID/LConn2
  x04_03_KT_L_001_1_RIGID/LConn2 -- x04_04_KB_L_001_1_RIGID/LConn6
  Transform/LConn1 -- ReferenceFrame/RConn1 -- Transform1/LConn1 -- Transform2/LConn1 -- Transform3/LConn1 -- Transform4/LConn1 -- Transform5/LConn1
  Parallel/LConn1 -- Transform/RConn1
  Parallel/RConn1 -- Transform1/RConn1
  Cartesian/LConn1 -- Transform2/RConn1
  Revolute1/LConn1 -- x04_05_BL_001_2_RIGID/RConn1
  Cartesian/RConn1 -- x04_03_KT_L_001_1_RIGID/LConn6
  x04_02_KB_R_001_1_RIGID/LConn1 -- x05_01_TI_R_001_1_RIGID/LConn2
  Cylindrical1/LConn1 -- x04_06_FL_001_1_RIGID/RConn1
  Cylindrical1/RConn1 -- x04_02_KB_R_001_1_RIGID/LConn2
  Revolute3/LConn1 -- x04_03_KT_L_001_1_RIGID/RConn1
  Revolute3/RConn1 -- x04_06_FL_001_2_RIGID/LConn2
  x03_01_FB_R_001_1_RIGID/LConn3 -- x03_02_FH_R_001_1_RIGID/LConn1
  Revolute4/LConn1 -- x04_01_KT_R_001_1_RIGID/RConn2
  Revolute4/RConn1 -- x04_05_BL_001_1_RIGID/LConn2
  x03_01_FB_R_001_1_RIGID/LConn4 -- x04_01_KT_R_001_1_RIGID/LConn1
  Revolute1/RConn1 -- x04_04_KB_L_001_1_RIGID/LConn7
  Cartesian1/LConn1 -- Transform3/RConn1
  Cartesian1/RConn1 -- x04_01_KT_R_001_1_RIGID/LConn2
  x04_01_KT_R_001_1_RIGID/LConn6 -- x04_02_KB_R_001_1_RIGID/LConn3
  Revolute5/LConn1 -- x04_01_KT_R_001_1_RIGID/RConn1
  Revolute5/RConn1 -- x04_06_FL_001_1_RIGID/LConn2
  Revolute6/LConn1 -- x6630T310_METRIC_BLACK_POLYPROPYLENE_BALL_KNOB_1_RIGID/RConn1
  Revolute6/RConn1 -- x92997A108_CORROSION_RESISTANT_SETUP_STUD_1_RIGID/LConn2
  Revolute7/LConn1 -- x92997A108_CORROSION_RESISTANT_SETUP_STUD_1_RIGID/RConn1
  Revolute7/RConn1 -- x03_02_FH_R_001_1_RIGID/LConn5
  Revolute8/LConn1 -- x6630T310_METRIC_BLACK_POLYPROPYLENE_BALL_KNOB_2_RIGID/RConn1
  Revolute2/LConn1 -- x04_03_KT_L_001_1_RIGID/RConn2
  Revolute8/RConn1 -- x92997A108_CORROSION_RESISTANT_SETUP_STUD_2_RIGID/LConn1
  Revolute9/LConn1 -- x92997A108_CORROSION_RESISTANT_SETUP_STUD_2_RIGID/RConn1
  Revolute9/RConn1 -- x03_04_FH_L_001_1_RIGID/LConn6
  x04_04_KB_L_001_1_RIGID/LConn3 -- F/RConn1
  x04_04_KB_L_001_1_RIGID/LConn4 -- F1/RConn1
  x04_04_KB_L_001_1_RIGID/LConn5 -- F2/RConn1
  x03_01_FB_R_001_1_RIGID/LConn1 -- F3/RConn1
  x03_01_FB_R_001_1_RIGID/LConn2 -- F4/RConn1
  x05_01_TI_R_001_1_RIGID/LConn1 -- F5/RConn1
  x04_02_KB_R_001_1_RIGID/LConn4 -- F6/RConn1
  Revolute2/RConn1 -- x04_05_BL_001_2_RIGID/LConn2
  x04_02_KB_R_001_1_RIGID/LConn5 -- F7/RConn1
  x04_02_KB_R_001_1_RIGID/LConn6 -- F8/RConn1
  x02_01_PE_001_1_RIGID/LConn12 -- F9/RConn1
  x02_01_PE_001_1_RIGID/LConn23 -- F10/RConn1
  x02_01_PE_001_1_RIGID/LConn24 -- F11/RConn1
  x02_01_PE_001_1_RIGID/LConn25 -- F12/RConn1
  x02_01_PE_001_1_RIGID/LConn26 -- F13/RConn1
  x02_01_PE_001_1_RIGID/LConn27 -- F14/RConn1
  x05_02_TI_001_1_RIGID/LConn1 -- F15/RConn1
  x02_01_PE_001_1_RIGID/LConn28 -- F16/RConn1
  x03_03_FB_L_001_1_RIGID/LConn1 -- x03_04_FH_L_001_1_RIGID/LConn5
  x02_01_PE_001_1_RIGID/LConn29 -- F17/RConn1
  x02_01_PE_001_1_RIGID/LConn2 -- F18/RConn1
  x02_01_PE_001_1_RIGID/LConn3 -- F19/RConn1
  x02_01_PE_001_1_RIGID/LConn4 -- F20/RConn1
  x02_01_PE_001_1_RIGID/LConn5 -- F21/RConn1
  x02_01_PE_001_1_RIGID/LConn6 -- F22/RConn1
  x02_01_PE_001_1_RIGID/LConn7 -- F23/RConn1
  x02_01_PE_001_1_RIGID/LConn8 -- F24/RConn1
  x02_01_PE_001_1_RIGID/LConn9 -- F25/RConn1
  x02_01_PE_001_1_RIGID/LConn10 -- F26/RConn1
  x03_03_FB_L_001_1_RIGID/LConn4 -- x04_03_KT_L_001_1_RIGID/LConn1
  x02_01_PE_001_1_RIGID/LConn11 -- F27/RConn1
  x02_01_PE_001_1_RIGID/LConn13 -- F28/RConn1
  x02_01_PE_001_1_RIGID/LConn14 -- F29/RConn1
  x02_01_PE_001_1_RIGID/LConn15 -- F30/RConn1
  x02_01_PE_001_1_RIGID/LConn16 -- F31/RConn1
  x02_01_PE_001_1_RIGID/LConn17 -- F32/RConn1
  x04_06_FL_001_1_RIGID/LConn1 -- F33/RConn1
  x04_06_FL_001_2_RIGID/LConn1 -- F34/RConn1
  x03_02_FH_R_001_1_RIGID/LConn2 -- F35/RConn1
  x92997A108_CORROSION_RESISTANT_SETUP_STUD_1_RIGID/LConn1 -- F36/RConn1
  x04_04_KB_L_001_1_RIGID/LConn1 -- x05_02_TI_001_1_RIGID/LConn2
  x03_04_FH_L_001_1_RIGID/LConn2 -- F37/RConn1
  x92997A108_CORROSION_RESISTANT_SETUP_STUD_2_RIGID/LConn2 -- F38/RConn1
  x03_04_FH_L_001_1_RIGID/LConn3 -- F39/RConn1
  x03_04_FH_L_001_1_RIGID/LConn4 -- F40/RConn1
  x04_03_KT_L_001_1_RIGID/LConn3 -- F41/RConn1
  x04_03_KT_L_001_1_RIGID/LConn4 -- F42/RConn1
  x04_03_KT_L_001_1_RIGID/LConn5 -- F43/RConn1
  x04_01_KT_R_001_1_RIGID/LConn3 -- F44/RConn1
  x04_01_KT_R_001_1_RIGID/LConn4 -- F45/RConn1
  x03_02_FH_R_001_1_RIGID/LConn3 -- F46/RConn1
  Spherical/LConn1 -- x02_01_PE_001_1_RIGID/RConn2
  x03_02_FH_R_001_1_RIGID/LConn4 -- F47/RConn1
  x04_01_KT_R_001_1_RIGID/LConn5 -- F48/RConn1
  x03_03_FB_L_001_1_RIGID/LConn2 -- F49/RConn1
  x03_03_FB_L_001_1_RIGID/LConn3 -- F50/RConn1
  x02_01_PE_001_1_RIGID/LConn18 -- F51/RConn1
  x02_01_PE_001_1_RIGID/LConn19 -- F52/RConn1
  x02_01_PE_001_1_RIGID/LConn20 -- F53/RConn1
  x02_01_PE_001_1_RIGID/LConn21 -- F54/RConn1
  x02_01_PE_001_1_RIGID/LConn22 -- F55/RConn1
  x04_05_BL_001_1_RIGID/LConn1 -- F56/RConn1

== system ah001_full_import/x90695A038_CLASS_04_STEEL_THIN_HEX_NUT_DIN_439B_1_RIGID ==
  ReferenceFrame : sm_lib/Frames and Transforms/Reference Frame
  Solid : sm_lib/Body Elements/File Solid  ExtGeomFileName=90695A038_CLASS 04 STEEL THIN HEX NUT - DIN 439B_90695A038_sldprt.STEP  UnitType=FromFile  ExtGeomFileUnits=m  StepReaderType=HEX  ExportConvexHullGeometry=off  InertiaType=Custom  BasedOnType=DensityFromFile  Density=1000  DensityUnits=kg/m^3  Mass=smiData.Solid(20).mass  MassUnits=kg  CenterOfMass=smiData.Solid(20).CoM  CenterOfMassUnits=mm  MomentsOfInertia=smiData.Solid(20).MoI  MomentsOfInertiaUnits=kg*mm^2  ProductsOfInertia=smiData.Solid(20).PoI  ProductsOfInertiaUnits=kg*mm^2  GraphicType=FromGeometry  MarkerShape=Sphere  MarkerSize=10  GraphicVisPropType=SimpleVisualProperties  GraphicDiffuseColor=smiData.Solid(20).color  GraphicOpacity=smiData.Solid(20).opacity  GraphicSpecularColor=[0.5 0.5 0.5 1.0]  GraphicAmbientColor=[0.15 0.15 0.15 1.0]  GraphicEmissiveColor=[0.0 0.0 0.0 1.0]  GraphicShininess=75  DoExposeReferenceFrame=on  SerializedFrames=<Frames/>
  Transform : sm_lib/Frames and Transforms/Rigid Transform  RotationMethod=ArbitraryAxis  FollAlignAxisA=+X  BaseAlignAxisA=+Y  FollAlignAxisB=+Y  BaseAlignAxisB=+Z  RotationStandardAxis=+Z  RotationAngle=smiData.RigidTransform(122).angle  RotationAngleUnits=rad  RotationArbitraryAxis=smiData.RigidTransform(122).axis  RotationSequenceAxes=FollowerAxes  RotationSequence=XYX  RotationSequenceAngles=[0 0 0]  RotationSequenceAnglesUnits=deg  RotationMatrix=[1 0 0;0 1 0;0 0 1]  Quaternion=[1 0 0 0]  TranslationMethod=Cartesian  TranslationCartesianOffset=smiData.RigidTransform(122).translation  TranslationCartesianOffsetUnits=mm  TranslationStandardAxis=+Z  TranslationStandardOffset=0  TranslationStandardOffsetUnits=m  TranslationROffset=0  TranslationROffsetUnits=m  TranslationThetaOffset=0  TranslationThetaOffsetUnits=deg  TranslationZOffset=0  TranslationZOffsetUnits=m
  Transform1 : sm_lib/Frames and Transforms/Rigid Transform  RotationMethod=ArbitraryAxis  FollAlignAxisA=+X  BaseAlignAxisA=+Y  FollAlignAxisB=+Y  BaseAlignAxisB=+Z  RotationStandardAxis=+Z  RotationAngle=smiData.RigidTransform(124).angle  RotationAngleUnits=rad  RotationArbitraryAxis=smiData.RigidTransform(124).axis  RotationSequenceAxes=FollowerAxes  RotationSequence=XYX  RotationSequenceAngles=[0 0 0]  RotationSequenceAnglesUnits=deg  RotationMatrix=[1 0 0;0 1 0;0 0 1]  Quaternion=[1 0 0 0]  TranslationMethod=Cartesian  TranslationCartesianOffset=smiData.RigidTransform(124).translation  TranslationCartesianOffsetUnits=mm  TranslationStandardAxis=+Z  TranslationStandardOffset=0  TranslationStandardOffsetUnits=m  TranslationROffset=0  TranslationROffsetUnits=m  TranslationThetaOffset=0  TranslationThetaOffsetUnits=deg  TranslationZOffset=0  TranslationZOffsetUnits=m
  F1 : PMIOPort  Side=Left
  F : PMIOPort  Port=2  Side=Left
  connections:
  Solid/RConn1 -- ReferenceFrame/RConn1 -- Transform/LConn1 -- Transform1/LConn1
  Transform/RConn1 -- F/RConn1
  Transform1/RConn1 -- F1/RConn1
